simulink model "psm_sv_ekf_bemf_ctrl"  (R2026a)
settings: Solver=ode23tb  StopTime=simlength  FixedStep=tc  MaxStep=tc
values from neighbouring files (symbols this model uses):
  A1_tilde_ekf = [-Rs_norm/Lalpha_norm 0 0 0 0 0; 0 -Rs_norm/Lalpha_norm 0 0 0 0;      0 0 0 0 0 0; 0 0 0 0 0 0;      0 0 0 0 0 1; 0 0 0 0 0 0]    [kalman_psm.m]
  A2_tilde_ekf = [0 0 0 1/Lbeta_norm 0 0; 0 0 -1/Lbeta_norm 0 0 0;      0 0 0 -1 0 0; 0 0 1 0 0 0;     0 0 0 0 0 0; 0 0 0 0 0 0]    [kalman_psm.m]
  A3_tilde_ekf = [0 0 0 0 0 0; 0 0 0 0 0 -1/Lbeta_norm;      0 0 0 0 0 0; 0 0 0 0 0 1;     0 0 0 0 0 0; 0 0 0 0 0 0]    [kalman_psm.m]
  A4_tilde_ekf = [0 0 0 0 0 1/Lalpha_norm; 0 0 0 0 0 0;      0 0 0 0 0 -1; 0 0 0 0 0 0;     0 0 0 0 0 0; 0 0 0 0 0 0]    [kalman_psm.m]
  Bd_ekf = B_tilde_ekf*ts_inv    [kalman_psm.m]
  C_ekf = [1 0 0 0 0 0; 0 1 0 0 0 0]    [kalman_psm.m]
  CTRPIFF_CLIP_RELEASE = 0.001    [init_model.m]
  dead_time_INV = 3e-6    (= 3e-06)    [init_model.m]
  fPWM_INV = fPWM_AFE    (= 5000)    [init_model.m]
  g0_10Hz = fcut_10Hz_flt * ts_afe * 2*pi    (= 0.0125663706144)    [init_model.m]
  g0_1Hz = fcut_1Hz_flt * ts_afe * 2*pi    (= 0.00125663706144)    [init_model.m]
  g1_10Hz = 1 - g0_10Hz    (= 0.987433629386)    [init_model.m]
  g1_1Hz = 1 - g0_1Hz    (= 0.998743362939)    [init_model.m]
  id_lim = 0.35    [init_model.m]
  inv_m_scale = motorc_m_scale    [init_model.m]
  iq_lim = 1.4    [init_model.m]
  kg = Kobs(1)    [init_model.m]
  ki_align = 0.1    [init_model.m]
  ki_i = 18    [init_model.m]
  ki_w = 8    [init_model.m]
  kp_align = 0.6    [init_model.m]
  kp_i = 0.25    [init_model.m]
  kp_w = 2    [init_model.m]
  kw = Kobs(2)    [init_model.m]
  lim_down_align = -0.2    [init_model.m]
  lim_up_align = 0.2    [init_model.m]
  number_of_modules = 1    [init_model.m]
  omega_m_sim = omega_m_bez    [init_model.m]
  Qkalman = ts_inv * [Rs_norm/Lalpha_norm 0 0 0 0 0; 0 Rs_norm/Lbeta_norm 0 0 0 0;      0 0 1 0 0 0;     0 0 0 1 0 0;     0 0 0 0 1 0;     0 0 0 0 0 1]    [kalman_psm.m]
  Rkalman = [ts_inv 0; 0 ts_inv]    [kalman_psm.m]
  simlength = 2    [init_model.m]
  tc = ts_afe/100    (= 2e-06)    [init_model.m]
  time_gain_afe_module_1 = 1.0    (= 1)    [init_model.m]
  time_gain_inv_module_2 = 1.0    (= 1)    [init_model.m]
  time_start_motor_control = 0.025    [init_model.m]
  ts_inv = 1/fPWM_INV    (= 0.0002)    [init_model.m]
undefined symbols (not defined in the file or in its folder): ibez, La, Lb, Ld_norm, Lq_norm, magnitude, omega_bez, omega_m_bez, psi_bez, psi_m, rpm_base, rpm_bez, Rs, tau_bez, torque_base, ubez
libraries: fl_lib x24, nesl_utility x11, cstblocks_lti x2, single_phase_pwm_modulator x1, threephase_inductor_lib x1, simple_flexible_shaft x1, permanent_magnet_synchronous_machine x1
(part 2 of 2)

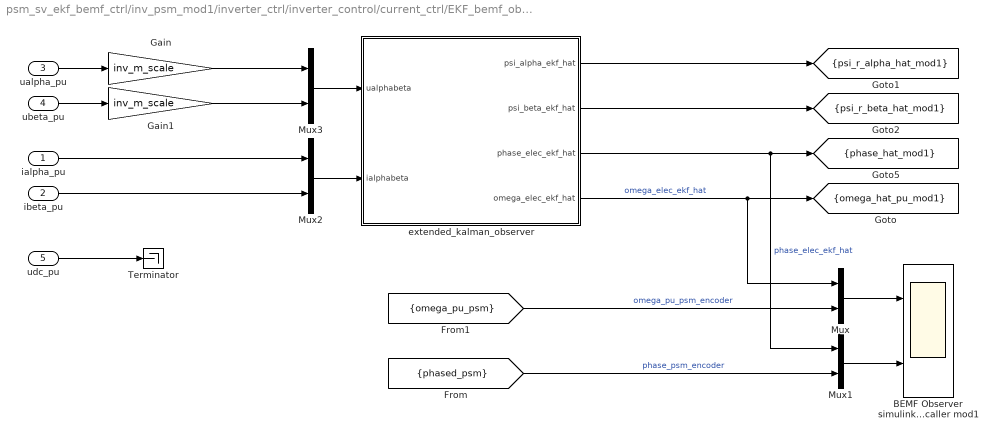
== system psm_sv_ekf_bemf_ctrl/inv_psm_mod1/inverter_ctrl/inverter_control/current_ctrl/EKF_bemf_observer ==
  ialpha_pu : Inport
  ibeta_pu : Inport  Port=2
  ualpha_pu : Inport  Port=3
  ubeta_pu : Inport  Port=4
  udc_pu : Inport  Port=5
  BEMF Observer simulink/Ccaller mod1 : Scope  NumInputPorts=2
      settings: ActiveDisplayYMinimum=-3.9268288357338932  ActiveDisplayYMaximum=3.9255329857071075
  Gain : Gain  Gain=inv_m_scale
  Gain1 : Gain  Gain=inv_m_scale
  Mux{,1..3} (4 alike) : Mux  Inputs=2
  Terminator : Terminator
  extended_kalman_observer : Subsystem
  tag scope: omega_hat_pu_mod1=scoped, phase_hat_mod1=scoped, psi_r_alpha_hat_mod1=scoped, psi_r_beta_hat_mod1=scoped
  wires:
  ialpha_pu/1 -> Mux2/1
  ibeta_pu/1 -> Mux2/2
  Mux/1 -> BEMF Observer simulink/Ccaller mod1/1
  Mux1/1 -> BEMF Observer simulink/Ccaller mod1/2
  ualpha_pu/1 -> Gain/1
  ubeta_pu/1 -> Gain1/1
  extended_kalman_observer/3(phase_elec_ekf_hat) -> [phase_hat_mod1], Mux1/1  "phase_elec_ekf_hat"
  extended_kalman_observer/4(omega_elec_ekf_hat) -> Mux/1, [omega_hat_pu_mod1]  "omega_elec_ekf_hat"
  [omega_pu_psm] -> Mux/2  "omega_pu_psm_encoder"
  [phased_psm] -> Mux1/2  "phase_psm_encoder"
  udc_pu/1 -> Terminator/1
  extended_kalman_observer/1(psi_alpha_ekf_hat) -> [psi_r_alpha_hat_mod1]
  extended_kalman_observer/2(psi_beta_ekf_hat) -> [psi_r_beta_hat_mod1]
  Mux2/1 -> extended_kalman_observer/2(ialphabeta)
  Mux3/1 -> extended_kalman_observer/1(ualphabeta)
  Gain/1 -> Mux3/1
  Gain1/1 -> Mux3/2

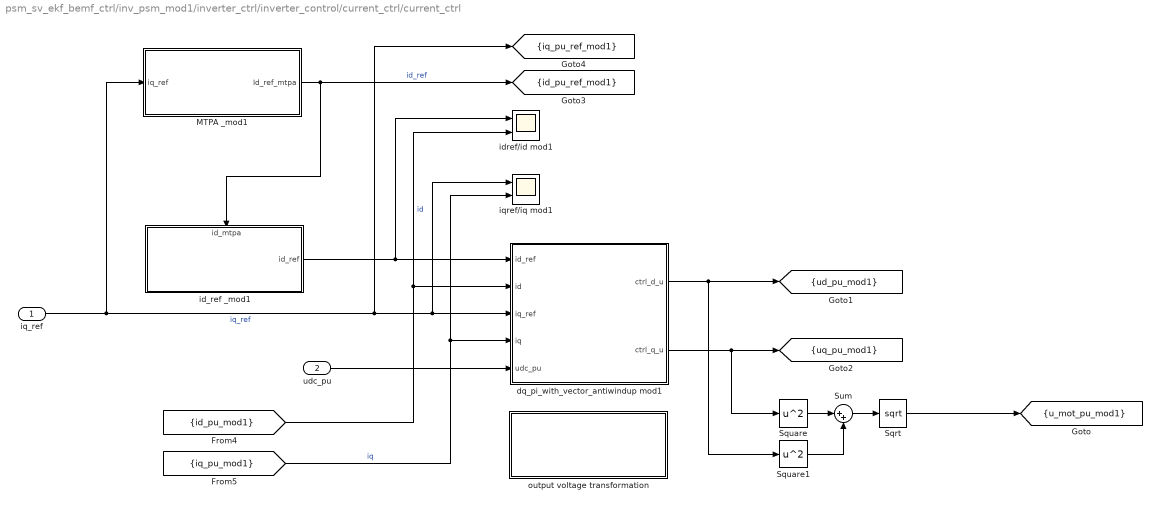
== system psm_sv_ekf_bemf_ctrl/inv_psm_mod1/inverter_ctrl/inverter_control/current_ctrl/current_ctrl ==
  iq_ref : Inport
  udc_pu : Inport  Port=2
  MTPA _mod1 : Subsystem
  Sqrt : Sqrt
  Square : Math  Operator=square
  Square1 : Math  Operator=square
  Sum : Sum  Inputs=|++
  dq_pi_with_vector_antiwindup mod1 : Subsystem
  id_ref _mod1 : Subsystem
      settings: PortSchema="{\"entries\":[{\"content\":{\"sides\":[{\"content\":{},\"type\":\"ConnectorPlacement.EquallySpacedRectSide\",\"uuid\":\"42af5d69-f0eb-42c6-9e03-28c1d0757323\"},{\"content\":{\"connectorIds\":[\"Out1\"],\"side\":\"RIGHT\"},\"type\":\"ConnectorPlacement.EquallySpacedRectSide\",\"uuid\":\"dd68a9f9-d15f-4e57-9d9e-130889a7b90c\"},{\"content\":{\"connectorIds\":[\"In1\"],\"side\":\"TOP\"},\"type\":\"ConnectorPlacement.EquallySpacedRectSide\",\"uuid\":\"68c797a2-8439-4b8d-8368-b7485adf0676\"}]},\"type\":\"ConnectorPlacement.EquallySpacedConnector\",\"uuid\":\"693c5f1c-0580-4626-8f13-b27865dfb3ac\"}],\"packageUris\":[\"http://schema.mathworks.com/mf0/Connector/R2020b\"],\"version\":\"1.0\"}"
  idref/id mod1 : Scope  NumInputPorts=2
      settings: ActiveDisplayYMinimum=-0.6792366431007606  ActiveDisplayYMaximum=0.075577635851628425
  iqref/iq mod1 : Scope  NumInputPorts=2
      settings: ActiveDisplayYMinimum=-2.4850184275737042  ActiveDisplayYMaximum=0.33436168402982208  DataLoggingVariableName=ScopeData2
  output voltage transformation : Subsystem
  tag scope: id_pu_ref_mod1=scoped, iq_pu_ref_mod1=scoped, u_mot_pu_mod1=scoped, ud_pu_mod1=scoped, uq_pu_mod1=scoped
  wires:
  [iq_pu_mod1] -> iqref/iq mod1/2, dq_pi_with_vector_antiwindup mod1/4(iq)  "iq"
  [id_pu_mod1] -> idref/id mod1/2, dq_pi_with_vector_antiwindup mod1/2(id)  "id"
  MTPA _mod1/1(Id_ref_mtpa) -> id_ref _mod1/1(id_mtpa), [id_pu_ref_mod1]  "id_ref"
  iq_ref/1 -> MTPA _mod1/1(iq_ref), iqref/iq mod1/1, dq_pi_with_vector_antiwindup mod1/3(iq_ref), [iq_pu_ref_mod1]  "iq_ref"
  dq_pi_with_vector_antiwindup mod1/1(ctrl_d_u) -> [ud_pu_mod1], Square1/1
  dq_pi_with_vector_antiwindup mod1/2(ctrl_q_u) -> [uq_pu_mod1], Square/1
  Square/1 -> Sum/1
  Sum/1 -> Sqrt/1
  Square1/1 -> Sum/2
  Sqrt/1 -> [u_mot_pu_mod1]
  id_ref _mod1/1(id_ref) -> idref/id mod1/1, dq_pi_with_vector_antiwindup mod1/1(id_ref)
  udc_pu/1 -> dq_pi_with_vector_antiwindup mod1/5(udc_pu)

== system psm_sv_ekf_bemf_ctrl/inv_psm_mod1/inverter_ctrl/inverter_control/current_ctrl/current_transformation ==
  Demux : Demux  Outputs=3
  alphabeta2dq : MATLAB Function  TreatAsAtomicUnit=on
  uvw2alphabeta : MATLAB Function  TreatAsAtomicUnit=on
  tag scope: ialpha_pu_mod1=scoped, ibeta_pu_mod1=scoped, id_pu_mod1=scoped, iq_pu_mod1=scoped
  wires:
  alphabeta2dq/2(q) -> [iq_pu_mod1]  "iq_pu"
  alphabeta2dq/1(d) -> [id_pu_mod1]  "id_pu"
  uvw2alphabeta/2(beta) -> alphabeta2dq/2(beta), [ibeta_pu_mod1]  "ibeta_pu"
  uvw2alphabeta/1(alpha) -> [ialpha_pu_mod1], alphabeta2dq/1(alpha)  "ialpha_pu"
  [motor_phase_ctrl_mod1] -> alphabeta2dq/3(gamma)
  Demux/3 -> uvw2alphabeta/3(w)  "iw"
  Demux/2 -> uvw2alphabeta/2(v)  "iv"
  Demux/1 -> uvw2alphabeta/1(u)  "iu"
  [isd_uvw_inv_mod1] -> Demux/1

== system psm_sv_ekf_bemf_ctrl/inv_psm_mod1/inverter_ctrl/inverter_control/encoder-sensorless-switch/double_integrator_observer ==
  phase_psm : Inport
  Dead Zone : DeadZone  LowerValue=-0.01  UpperValue=0.01
  Gain : Gain  Gain=kw
  Gain1 : Gain  Gain=kg
  Gain2 : Gain  Gain=omega_bez
  Gain3 : Gain  Gain=1/omega_bez
  Gain5 : Gain  Gain=ts_inv
  Sum : Sum  Inputs=-+|
  Sum1 : Sum  Inputs=|++
  Sum2 : Sum  Inputs=|++
  Sum8 : Sum  Inputs=++|
  Unit Delay1 : UnitDelay  InitialCondition=pi  SampleTime=-1
  Unit Delay2 : UnitDelay  SampleTime=-1
  bounder1 : MATLAB Function  TreatAsAtomicUnit=on
  bounder2 : MATLAB Function  TreatAsAtomicUnit=on
  phase_psm_hat : Outport  VectorParamsAs1DForOutWhenUnconnected=off
  omega_pu_psm_hat : Outport  Port=2  VectorParamsAs1DForOutWhenUnconnected=off
  wires:
  Gain1/1 -> Sum2/1
  phase_psm/1 -> Sum/2
  Sum8/1 -> Unit Delay1/1
  Unit Delay1/1 -> bounder2/1(u)
  Sum1/1 -> Unit Delay2/1
  Gain/1 -> Gain3/1
  Unit Delay2/1 -> omega_pu_psm_hat/1, Sum1/2, Gain5/1
  Sum2/1 -> Sum8/2
  bounder2/1(y) -> Sum2/2, phase_psm_hat/1, Sum/1  "phase_hat"
  bounder1/1(y) -> Gain1/1, Gain/1
  Gain2/1 -> Sum8/1
  Gain3/1 -> Sum1/1
  Gain5/1 -> Gain2/1
  Sum/1 -> bounder1/1(u)

== system psm_sv_ekf_bemf_ctrl/inv_psm_mod1/inverter_ctrl/inverter_control/is inv quantizzation and one step delay/is inv quantizzation and one step delay ==
  is_u_pu : Inport
  is_v_pu : Inport  Port=2
  is_w_pu : Inport  Port=3
  Gain3 : Gain  Gain=-1
  Gain4 : Gain  Gain=-1
  Gain5 : Gain  Gain=-1
  Quantizer : Quantizer  QuantizationInterval=adc_quantization
  Quantizer1 : Quantizer  QuantizationInterval=adc_quantization
  Quantizer2 : Quantizer  QuantizationInterval=adc_quantization
  Unit Delay : UnitDelay  SampleTime=-1
  Unit Delay1 : UnitDelay  SampleTime=-1
  Unit Delay2 : UnitDelay  SampleTime=-1
  Zero-Order Hold : ZeroOrderHold  SampleTime=-1
  Zero-Order Hold1 : ZeroOrderHold  SampleTime=-1
  Zero-Order Hold2 : ZeroOrderHold  SampleTime=-1
  isd_u_pu : Outport
  isd_v_pu : Outport  Port=2
  isd_w_pu : Outport  Port=3
  wires:
  Unit Delay/1 -> Gain3/1
  Unit Delay1/1 -> Gain4/1
  Unit Delay2/1 -> Gain5/1
  Quantizer/1 -> Unit Delay/1
  Quantizer1/1 -> Unit Delay1/1
  Quantizer2/1 -> Unit Delay2/1
  is_u_pu/1 -> Zero-Order Hold/1
  is_v_pu/1 -> Zero-Order Hold1/1
  is_w_pu/1 -> Zero-Order Hold2/1
  Gain3/1 -> isd_u_pu/1
  Gain4/1 -> isd_v_pu/1
  Gain5/1 -> isd_w_pu/1
  Zero-Order Hold/1 -> Quantizer/1
  Zero-Order Hold1/1 -> Quantizer1/1
  Zero-Order Hold2/1 -> Quantizer2/1

== system psm_sv_ekf_bemf_ctrl/inv_psm_mod1/inverter_ctrl/inverter_control/omega_pu/flt ==
  input : Inport
  Gain3 : Gain  Gain=g1_10Hz
  Gain6 : Gain  Gain=g0_10Hz
  Sum : Sum  Inputs=|++
  Unit Delay1 : UnitDelay  SampleTime=-1
  output : Outport  VectorParamsAs1DForOutWhenUnconnected=off
  wires:
  Gain6/1 -> Sum/1
  input/1 -> Gain6/1
  Unit Delay1/1 -> Gain3/1
  Gain3/1 -> Sum/2
  Sum/1 -> Unit Delay1/1, output/1

== system psm_sv_ekf_bemf_ctrl/inv_psm_mod1/inverter_ctrl/inverter_control/phase_compensation_1/alignment_ctrl ==
  local_time : Inport
  master_time : Inport  Port=2
  Constant : Constant  Value=0
  Gain : Gain  Gain=-1
  Sum : Sum  Inputs=|+-
  pi : Subsystem  mask{kp=kp_align, ki=ki_align, lim_up=lim_up_align, lim_down=lim_down_align}
      mask prompts: ki "ki*ts"
      mask Display:
      | disp('pi()');
      | port_label('input', 1, 'u_ref');
      | port_label('input', 2, 'u');
      | port_label('output', 1, 'y');
  dp : Outport
  wires:
  master_time/1 -> Sum/1
  Sum/1 -> Gain/1
  Constant/1 -> pi/1(u_ref)
  local_time/1 -> Sum/2
  Gain/1 -> pi/2(u)
  pi/1(y) -> dp/1

== system psm_sv_ekf_bemf_ctrl/inv_psm_mod1/inverter_ctrl/inverter_control/speed_reference_generator/flt ==
  input : Inport
  Gain3 : Gain  Gain=g1_1Hz
  Gain6 : Gain  Gain=g0_1Hz
  Sum : Sum  Inputs=|++
  Unit Delay1 : UnitDelay  SampleTime=-1
  output : Outport  VectorParamsAs1DForOutWhenUnconnected=off
  wires:
  Gain6/1 -> Sum/1
  input/1 -> Gain6/1
  Unit Delay1/1 -> Gain3/1
  Gain3/1 -> Sum/2
  Sum/1 -> Unit Delay1/1, output/1

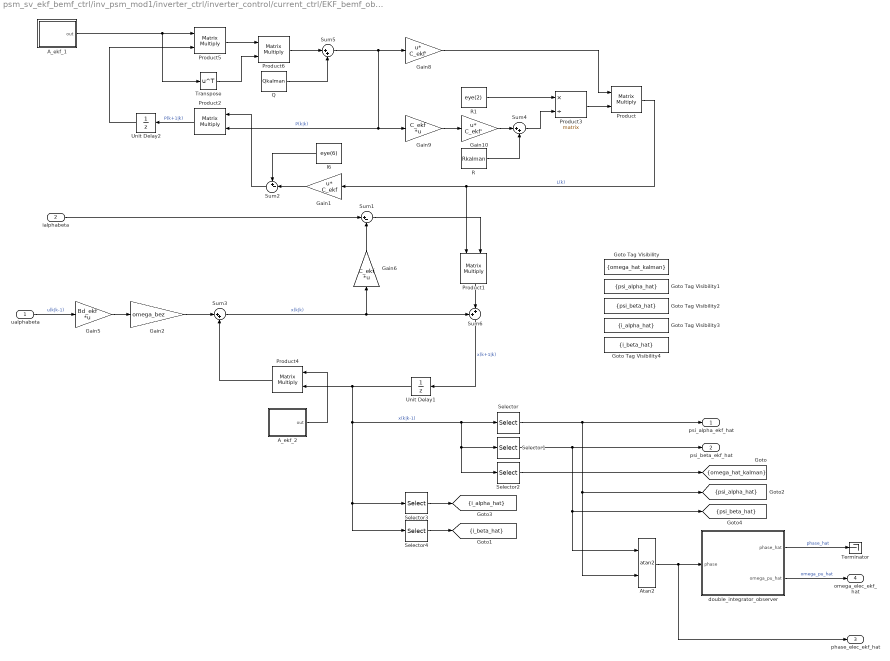
== system psm_sv_ekf_bemf_ctrl/inv_psm_mod1/inverter_ctrl/inverter_control/current_ctrl/EKF_bemf_observer/extended_kalman_observer ==
  ualphabeta : Inport
  ialphabeta : Inport  Port=2
  A_ekf_1 : Subsystem
  A_ekf_2 : Subsystem
  Atan2 : Trigonometry  Operator=atan2
  Gain1 : Gain  Gain=C_ekf  Multiplication=Matrix(u*K)
  Gain10 : Gain  Gain=C_ekf'  Multiplication=Matrix(u*K)
  Gain2 : Gain  Gain=omega_bez
  Gain5 : Gain  Gain=Bd_ekf  Multiplication=Matrix(K*u)
  Gain6 : Gain  Gain=C_ekf  Multiplication=Matrix(K*u)
  Gain8 : Gain  Gain=C_ekf'  Multiplication=Matrix(u*K)
  Gain9 : Gain  Gain=C_ekf  Multiplication=Matrix(K*u)
  Goto Tag Visibility : GotoTagVisibility  GotoTag=omega_hat_kalman
  Goto Tag Visibility1 : GotoTagVisibility  GotoTag=psi_alpha_hat
  Goto Tag Visibility2 : GotoTagVisibility  GotoTag=psi_beta_hat
  Goto Tag Visibility3 : GotoTagVisibility  GotoTag=i_alpha_hat
  Goto Tag Visibility4 : GotoTagVisibility  GotoTag=i_beta_hat
  I6 : Constant  Value=eye(6)
  Product{,1..2,4..6} (6 alike) : Product  Multiplication=Matrix(*)
  Product3 : Product  Inputs=*/  Multiplication=Matrix(*)
  Q : Constant  Value=Qkalman
  R : Constant  Value=Rkalman
  R1 : Constant  Value=eye(2)
  Selector : Selector  InputPortWidth=6  IndexOptions=Index vector (dialog)  Indices=3  OutputSizes=1
  Selector1 : Selector  InputPortWidth=6  IndexOptions=Index vector (dialog)  Indices=4  OutputSizes=1
  Selector2 : Selector  InputPortWidth=6  IndexOptions=Index vector (dialog)  Indices=6  OutputSizes=1
  Selector3 : Selector  InputPortWidth=6  IndexOptions=Index vector (dialog)  Indices=1  OutputSizes=1
  Selector4 : Selector  InputPortWidth=6  IndexOptions=Index vector (dialog)  Indices=2  OutputSizes=1
  Sum1 : Sum  Inputs=|+-
  Sum2 : Sum  Inputs=+-|
  Sum3 : Sum  Inputs=|++
  Sum4 : Sum  Inputs=|++
  Sum5 : Sum  Inputs=|++
  Sum6 : Sum  Inputs=++|
  Terminator : Terminator
  Transpose : Math  Operator=transpose
  Unit Delay1 : UnitDelay  InitialCondition=[0 0 1 1 0 0]*ts_inv  SampleTime=-1
  Unit Delay2 : UnitDelay  SampleTime=-1
  double_integrator_observer : Subsystem
  psi_alpha_ekf_hat : Outport
  psi_beta_ekf_hat : Outport  Port=2
  phase_elec_ekf_hat : Outport  Port=3
  omega_elec_ekf_hat : Outport  Port=4
  tag scope: i_alpha_hat=scoped, i_beta_hat=scoped, omega_hat_kalman=scoped, psi_alpha_hat=scoped, psi_beta_hat=scoped
  wires:
  Gain5/1 -> Gain2/1
  Gain6/1 -> Sum1/2
  Sum5/1 -> Gain8/1, Gain9/1, Product2/2  "P(k|k)"
  Product5/1 -> Product6/1
  Product6/1 -> Sum5/1
  Q/1 -> Sum5/2
  Gain9/1 -> Gain10/1
  R/1 -> Sum4/2
  Gain10/1 -> Sum4/1
  Gain8/1 -> Product/1
  Product/1 -> Product1/1, Gain1/1  "L(k)"
  Product2/1 -> Unit Delay2/1  "P(k+1|k)"
  Sum2/1 -> Product2/1
  Unit Delay2/1 -> Product5/2
  Sum6/1 -> Unit Delay1/1  "x(k+1|k)"
  I6/1 -> Sum2/1
  Gain1/1 -> Sum2/2
  Sum1/1 -> Product1/2
  ialphabeta/1 -> Sum1/1
  Sum4/1 -> Product3/2
  Product3/1 -> Product/2
  R1/1 -> Product3/1
  ualphabeta/1 -> Gain5/1  "u(k|k-1)"
  Sum3/1 -> Gain6/1, Sum6/1  "x(k|k)"
  Unit Delay1/1 -> Selector2/1, Selector1/1, Selector/1, Selector3/1, Selector4/1, Product4/2  "x(k|k-1)"
  A_ekf_2/1(out) -> Product4/1
  A_ekf_1/1(out) -> Transpose/1, Product5/1
  Product1/1 -> Sum6/2
  Selector1/1 -> Atan2/1, [psi_beta_hat], psi_beta_ekf_hat/1
  Selector/1 -> Atan2/2, [psi_alpha_hat], psi_alpha_ekf_hat/1
  Transpose/1 -> Product6/2
  Selector2/1 -> [omega_hat_kalman]
  Selector3/1 -> [i_alpha_hat]
  Selector4/1 -> [i_beta_hat]
  Product4/1 -> Sum3/2
  double_integrator_observer/2(omega_pu_hat) -> omega_elec_ekf_hat/1  "omega_pu_hat"
  Atan2/1 -> double_integrator_observer/1(phase), phase_elec_ekf_hat/1
  double_integrator_observer/1(phase_hat) -> Terminator/1  "phase_hat"
  Gain2/1 -> Sum3/1

== system psm_sv_ekf_bemf_ctrl/inv_psm_mod1/inverter_ctrl/inverter_control/current_ctrl/current_ctrl/MTPA _mod1 ==
  iq_ref : Inport
  Gain1 : Gain  Gain=1/(Ld_norm - Lq_norm)/2
  Gain2 : Gain  Gain=1/(Ld_norm - Lq_norm)/2
  Gain3 : Gain  Gain=-1
  Math Function1 : Math  Operator=magnitude^2  SignedPower=on
  Math Function4 : Math  Operator=magnitude^2  SignedPower=on
  Sqrt : Sqrt
  Sum : Sum  Inputs=|++
  Sum1 : Sum  Inputs=|-+
  id_ref_pu < x < 0 : Saturate  UpperLimit=0  LowerLimit=-id_lim
  Id_ref_mtpa : Outport  VectorParamsAs1DForOutWhenUnconnected=off
  wires:
  Sum1/1 -> Gain3/1
  id_ref_pu < x < 0/1 -> Id_ref_mtpa/1
  Math Function4/1 -> Sum/1
  Math Function1/1 -> Sum/2
  Gain1/1 -> Math Function4/1
  Sum/1 -> Sqrt/1
  Sqrt/1 -> Sum1/2
  iq_ref/1 -> Math Function1/1
  Gain2/1 -> Sum1/1
  [motor_speed_pu_ctrl_mod1] -> Gain1/1, Gain2/1
  Gain3/1 -> id_ref_pu < x < 0/1

== system psm_sv_ekf_bemf_ctrl/inv_psm_mod1/inverter_ctrl/inverter_control/current_ctrl/current_ctrl/dq_pi_with_vector_antiwindup mod1 ==
  id_ref : Inport
  id : Inport  Port=2
  iq_ref : Inport  Port=3
  iq : Inport  Port=4
  udc_pu : Inport  Port=5
  Variant Source : VariantSource  VariantControls={use_current_controller_from_simulink_module_1 == 1, use_current_controller_from_ccaller_module_1 == 1}
  Variant Source1 : VariantSource  VariantControls={use_current_controller_from_simulink_module_1 == 1, use_current_controller_from_ccaller_module_1 == 1}
  dq_vector_pi : Subsystem
  dq_vector_pi_ccaller : Subsystem
  simulink/Ccaller VectorPI : Scope  NumInputPorts=2
      settings: ActiveDisplayYMinimum=-1.0778845462482423  ActiveDisplayYMaximum=0.14052729005925355
  ctrl_d_u : Outport
  ctrl_q_u : Outport  Port=2
  wires:
  id/1 -> dq_vector_pi_ccaller/1(id), dq_vector_pi/1(id)  "id"
  id_ref/1 -> dq_vector_pi_ccaller/2(id_ref), dq_vector_pi/2(id_ref)  "id_ref"
  iq/1 -> dq_vector_pi_ccaller/3(iq), dq_vector_pi/3(iq)  "iq"
  iq_ref/1 -> dq_vector_pi_ccaller/4(iq_ref), dq_vector_pi/4(iq_ref)  "iq_ref"
  dq_vector_pi/1(md_sat) -> Variant Source/1
  dq_vector_pi_ccaller/2(uq_ctrl_out) -> Variant Source1/2
  dq_vector_pi/2(mq_sat) -> Variant Source1/1
  dq_vector_pi_ccaller/1(ud_ctrl_out) -> Variant Source/2
  Variant Source/1 -> ctrl_d_u/1, simulink/Ccaller VectorPI/1  "ctrl_d_u"
  Variant Source1/1 -> simulink/Ccaller VectorPI/2, ctrl_q_u/1  "ctrl_q_u"
  udc_pu/1 -> dq_vector_pi_ccaller/5(udc_pu)

== system psm_sv_ekf_bemf_ctrl/inv_psm_mod1/inverter_ctrl/inverter_control/current_ctrl/current_ctrl/id_ref _mod1 ==
  id_mtpa : Inport
  Constant : Constant  Value=0
  Variant Source : VariantSource  VariantControls={use_mtpa == 1, use_mtpa == 0}
  id_ref : Outport
  wires:
  Variant Source/1 -> id_ref/1
  id_mtpa/1 -> Variant Source/1
  Constant/1 -> Variant Source/2

== system psm_sv_ekf_bemf_ctrl/inv_psm_mod1/inverter_ctrl/inverter_control/current_ctrl/current_ctrl/output voltage transformation ==
  Unit Delay2 : UnitDelay  SampleTime=-1
  Unit Delay3 : UnitDelay  SampleTime=-1
  dq2alphabeta : MATLAB Function  TreatAsAtomicUnit=on
  tag scope: ualpha_pu_mod1=scoped, ubeta_pu_mod1=scoped
  wires:
  [ud_pu_mod1] -> dq2alphabeta/1(d)
  [uq_pu_mod1] -> dq2alphabeta/2(q)
  Unit Delay2/1 -> [ualpha_pu_mod1]
  dq2alphabeta/2(beta) -> Unit Delay3/1
  Unit Delay3/1 -> [ubeta_pu_mod1]
  dq2alphabeta/1(alpha) -> Unit Delay2/1
  [motor_phase_ctrl_mod1] -> dq2alphabeta/3(gamma)

== system psm_sv_ekf_bemf_ctrl/inv_psm_mod1/inverter_ctrl/inverter_control/phase_compensation_1/alignment_ctrl/pi ==
  u_ref : Inport
  u : Inport  Port=2
  1/Ti : Gain  Gain=kp  SaturateOnIntegerOverflow=on  OutDataTypeStr=Inherit: Same as input  ParamDataTypeStr=Inherit: Same as input
  Saturation : Saturate  UpperLimit=lim_up  LowerLimit=lim_down
  Sum1 : Sum  Inputs=+++  SaturateOnIntegerOverflow=on
  Sum2 : Sum  Inputs=-+  SaturateOnIntegerOverflow=on
  Sum3 : Sum  Inputs=-+  SaturateOnIntegerOverflow=on
  Unit Delay4 : UnitDelay  SampleTime=-1
  kp : Gain  Gain=ki  SaturateOnIntegerOverflow=on  OutDataTypeStr=Inherit: Same as input  ParamDataTypeStr=Inherit: Same as input
  y : Outport
  wires:
  1/Ti/1 -> Sum1/1, Sum3/1
  kp/1 -> Sum1/2
  Sum3/1 -> Unit Delay4/1
  Unit Delay4/1 -> Sum1/3
  u_ref/1 -> Sum2/2
  u/1 -> Sum2/1
  Sum2/1 -> kp/1, 1/Ti/1
  Sum1/1 -> Saturation/1
  Saturation/1 -> Sum3/2, y/1

== system psm_sv_ekf_bemf_ctrl/inv_psm_mod1/inverter_ctrl/inverter_control/current_ctrl/EKF_bemf_observer/extended_kalman_observer/A_ekf_1 ==
  Gain1 : Gain  Gain=A2_tilde_ekf
  Gain{7..10} (4 alike) : Gain  Gain=omega_bez
  Gain{2,4,6,11} (4 alike) : Gain  Gain=ts_inv
  Gain3 : Gain  Gain=A3_tilde_ekf
  Gain5 : Gain  Gain=A4_tilde_ekf
  I1 : Constant  Value=eye(6)
  I2 : Constant  Value=A1_tilde_ekf
  Sum7 : Sum  Inputs=+++++
  out : Outport
  wires:
  [psi_beta_hat] -> Gain5/1
  [psi_alpha_hat] -> Gain3/1
  [omega_hat_kalman] -> Gain1/1
  Gain5/1 -> Gain6/1
  Gain3/1 -> Gain4/1
  Gain1/1 -> Gain2/1
  I1/1 -> Sum7/1
  I2/1 -> Gain11/1
  Sum7/1 -> out/1
  Gain11/1 -> Gain7/1
  Gain2/1 -> Gain8/1
  Gain4/1 -> Gain9/1
  Gain6/1 -> Gain10/1
  Gain7/1 -> Sum7/2
  Gain8/1 -> Sum7/3
  Gain9/1 -> Sum7/4
  Gain10/1 -> Sum7/5

== system psm_sv_ekf_bemf_ctrl/inv_psm_mod1/inverter_ctrl/inverter_control/current_ctrl/EKF_bemf_observer/extended_kalman_observer/A_ekf_2 ==
  Gain1 : Gain  Gain=A2_tilde_ekf
  Gain{7..10} (4 alike) : Gain  Gain=omega_bez
  Gain{2,4,6,11} (4 alike) : Gain  Gain=ts_inv
  Gain3 : Gain  Gain=A3_tilde_ekf
  Gain5 : Gain  Gain=A4_tilde_ekf
  I1 : Constant  Value=eye(6)
  I2 : Constant  Value=A1_tilde_ekf
  Sum7 : Sum  Inputs=+++++
  out : Outport
  wires:
  Sum7/1 -> out/1
  I2/1 -> Gain11/1
  I1/1 -> Sum7/1
  Gain1/1 -> Gain2/1
  Gain3/1 -> Gain4/1
  Gain5/1 -> Gain6/1
  [omega_hat_kalman] -> Gain1/1
  [psi_alpha_hat] -> Gain3/1
  [psi_beta_hat] -> Gain5/1
  Gain11/1 -> Gain7/1
  Gain2/1 -> Gain8/1
  Gain4/1 -> Gain9/1
  Gain6/1 -> Gain10/1
  Gain7/1 -> Sum7/2
  Gain8/1 -> Sum7/3
  Gain9/1 -> Sum7/4
  Gain10/1 -> Sum7/5

== system psm_sv_ekf_bemf_ctrl/inv_psm_mod1/inverter_ctrl/inverter_control/current_ctrl/EKF_bemf_observer/extended_kalman_observer/double_integrator_observer ==
  phase : Inport
  Dead Zone : DeadZone  LowerValue=-0.01  UpperValue=0.01
  Gain : Gain  Gain=kw
  Gain1 : Gain  Gain=kg
  Gain2 : Gain  Gain=omega_bez
  Gain3 : Gain  Gain=1/omega_bez
  Gain5 : Gain  Gain=ts_inv
  Sum : Sum  Inputs=-+|
  Sum1 : Sum  Inputs=|++
  Sum2 : Sum  Inputs=|++
  Sum8 : Sum  Inputs=++|
  Unit Delay1 : UnitDelay  InitialCondition=pi  SampleTime=-1
  Unit Delay2 : UnitDelay  SampleTime=-1
  bounder1 : MATLAB Function  TreatAsAtomicUnit=on
  bounder2 : MATLAB Function  TreatAsAtomicUnit=on
  phase_hat : Outport  VectorParamsAs1DForOutWhenUnconnected=off
  omega_pu_hat : Outport  Port=2  VectorParamsAs1DForOutWhenUnconnected=off
  wires:
  Gain1/1 -> Sum2/1
  phase/1 -> Sum/2
  Sum8/1 -> Unit Delay1/1
  Unit Delay1/1 -> bounder2/1(u)
  Sum1/1 -> Unit Delay2/1
  Gain/1 -> Gain3/1
  Unit Delay2/1 -> omega_pu_hat/1, Sum1/2, Gain5/1
  Sum2/1 -> Sum8/2
  bounder2/1(y) -> Sum2/2, phase_hat/1, Sum/1  "phase_hat"
  bounder1/1(y) -> Gain1/1, Gain/1
  Gain2/1 -> Sum8/1
  Gain3/1 -> Sum1/1
  Gain5/1 -> Gain2/1
  Sum/1 -> bounder1/1(u)

== system psm_sv_ekf_bemf_ctrl/inv_psm_mod1/inverter_ctrl/inverter_control/current_ctrl/current_ctrl/dq_pi_with_vector_antiwindup mod1/dq_vector_pi ==
  id : Inport
  id_ref : Inport  Port=2
  iq : Inport  Port=3
  iq_ref : Inport  Port=4
  Sum1 : Sum  Inputs=|-+
  Sum2 : Sum  Inputs=|-+
  bounder1 : Subsystem
  bounder2 : Subsystem
  pi_d : Subsystem
  pi_q : Subsystem
  switch : Subsystem
  vector lenght : Subsystem
  md_sat : Outport
  mq_sat : Outport  Port=2
  wires:
  bounder2/2(clip) -> switch/2(clip 2)
  vector lenght/2(m) -> bounder1/3(m), bounder2/1(m)
  Sum2/1 -> pi_q/1(iq_tilde)
  pi_d/1(ud_out) -> vector lenght/1(md), bounder1/1(md)
  pi_q/1(Vqs_out) -> bounder2/3(mq), vector lenght/2(mq)
  vector lenght/1(m_1) -> bounder1/2(m_1), bounder2/2(m_1)
  switch/1(clip) -> pi_q/2(clip), pi_d/2(clip)
  iq/1 -> Sum2/1
  Sum1/1 -> pi_d/1(id_tilde)
  bounder1/2(clip) -> switch/1(clip 1)
  id/1 -> Sum1/1
  bounder1/1(md_sat) -> md_sat/1
  bounder2/1(mq_sat) -> mq_sat/1
  id_ref/1 -> Sum1/2
  iq_ref/1 -> Sum2/2

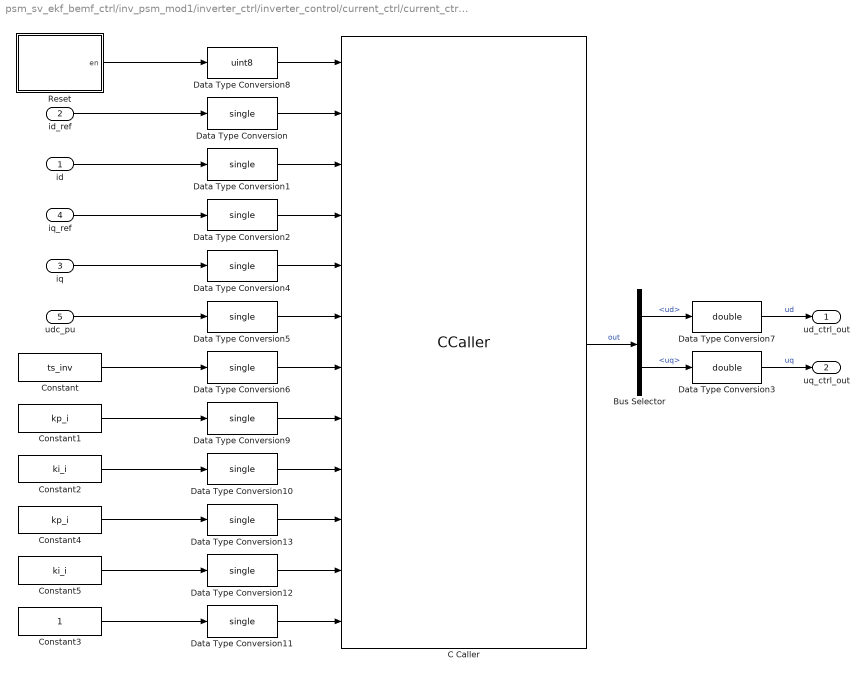
== system psm_sv_ekf_bemf_ctrl/inv_psm_mod1/inverter_ctrl/inverter_control/current_ctrl/current_ctrl/dq_pi_with_vector_antiwindup mod1/dq_vector_pi_ccaller ==
  id : Inport
  id_ref : Inport  Port=2
  iq : Inport  Port=3
  iq_ref : Inport  Port=4
  udc_pu : Inport  Port=5
  Bus Selector : BusSelector  OutputSignals=ud,uq
  C Caller : CCaller  FunctionName=dqvector_pi_process_simulink  PortSpecificationStruct="%)30     .    ,!8   8    (     @         %    \"     T    !     0         %  0 \"0    $    _    07)G3F%M90  4&]R=$YA;64 4V-O<&4     26YD97@     5'EP90      4VEZ90      27-';&]B86P   X    P    !@    @    $          4    (     0    ,    !         !   P!O=70 #@   #     &    \"     0         !0    @    !     P    $         $  # &]U=  .    .     8    (    !          %    \"     $    &     0         0   ...(+7280 chars)"
  Constant : Constant  Value=ts_inv
  Constant1 : Constant  Value=kp_i
  Constant2 : Constant  Value=ki_i
  Constant3 : Constant
  Constant4 : Constant  Value=kp_i
  Constant5 : Constant  Value=ki_i
  Data Type Conversion{,1..2,4..6,9..13} (11 alike) : DataTypeConversion  OutDataTypeStr=single  SaturateOnIntegerOverflow=off  RndMeth=Floor
  Data Type Conversion3 : DataTypeConversion  OutDataTypeStr=double  SaturateOnIntegerOverflow=off  RndMeth=Floor
  Data Type Conversion7 : DataTypeConversion  OutDataTypeStr=double  SaturateOnIntegerOverflow=off  RndMeth=Floor
  Data Type Conversion8 : DataTypeConversion  OutDataTypeStr=uint8  SaturateOnIntegerOverflow=off  RndMeth=Floor
  Reset : Subsystem
  ud_ctrl_out : Outport
  uq_ctrl_out : Outport  Port=2
  wires:
  Data Type Conversion5/1 -> C Caller/6
  Data Type Conversion/1 -> C Caller/2
  C Caller/1 -> Bus Selector/1  "out"
  Data Type Conversion1/1 -> C Caller/3
  Data Type Conversion4/1 -> C Caller/5
  Data Type Conversion2/1 -> C Caller/4
  Data Type Conversion6/1 -> C Caller/7
  Bus Selector/2 -> Data Type Conversion3/1  "<uq>"
  Bus Selector/1 -> Data Type Conversion7/1  "<ud>"
  Data Type Conversion7/1 -> ud_ctrl_out/1  "ud"
  Data Type Conversion3/1 -> uq_ctrl_out/1  "uq"
  Data Type Conversion8/1 -> C Caller/1
  Data Type Conversion9/1 -> C Caller/8
  Data Type Conversion10/1 -> C Caller/9
  Data Type Conversion11/1 -> C Caller/12
  Data Type Conversion13/1 -> C Caller/10
  Data Type Conversion12/1 -> C Caller/11
  Constant3/1 -> Data Type Conversion11/1
  Constant5/1 -> Data Type Conversion12/1
  Constant4/1 -> Data Type Conversion13/1
  Constant2/1 -> Data Type Conversion10/1
  Constant1/1 -> Data Type Conversion9/1
  Constant/1 -> Data Type Conversion6/1
  udc_pu/1 -> Data Type Conversion5/1
  iq/1 -> Data Type Conversion4/1
  iq_ref/1 -> Data Type Conversion2/1
  Reset/1(en) -> Data Type Conversion8/1
  id_ref/1 -> Data Type Conversion/1
  id/1 -> Data Type Conversion1/1

== system psm_sv_ekf_bemf_ctrl/inv_psm_mod1/inverter_ctrl/inverter_control/current_ctrl/current_ctrl/dq_pi_with_vector_antiwindup mod1/dq_vector_pi/bounder1 ==
  md : Inport
  m_1 : Inport  Port=2
  m : Inport  Port=3
  Constant : Constant
  Constant1 : Constant  Value=0
  Divide : Product
  Switch : Switch  Threshold=1  SaturateOnIntegerOverflow=off  InputSameDT=off
  Switch1 : Switch  Threshold=1  SaturateOnIntegerOverflow=off  InputSameDT=off
  md_sat : Outport  VectorParamsAs1DForOutWhenUnconnected=off
  clip : Outport  Port=2  VectorParamsAs1DForOutWhenUnconnected=off
  wires:
  md/1 -> Switch1/3, Divide/2
  m_1/1 -> Divide/1
  Divide/1 -> Switch1/1
  Switch1/1 -> md_sat/1
  Switch/1 -> clip/1
  m/1 -> Switch/2, Switch1/2
  Constant/1 -> Switch/1
  Constant1/1 -> Switch/3

== system psm_sv_ekf_bemf_ctrl/inv_psm_mod1/inverter_ctrl/inverter_control/current_ctrl/current_ctrl/dq_pi_with_vector_antiwindup mod1/dq_vector_pi/bounder2 ==
  m : Inport
  m_1 : Inport  Port=2
  mq : Inport  Port=3
  Constant : Constant
  Constant1 : Constant  Value=0
  Divide : Product
  Switch : Switch  Threshold=1  SaturateOnIntegerOverflow=off  InputSameDT=off
  Switch1 : Switch  Threshold=1  SaturateOnIntegerOverflow=off  InputSameDT=off
  mq_sat : Outport  VectorParamsAs1DForOutWhenUnconnected=off
  clip : Outport  Port=2  VectorParamsAs1DForOutWhenUnconnected=off
  wires:
  Constant1/1 -> Switch/3
  Constant/1 -> Switch/1
  m/1 -> Switch1/2, Switch/2
  Switch/1 -> clip/1
  Switch1/1 -> mq_sat/1
  Divide/1 -> Switch1/1
  m_1/1 -> Divide/1
  mq/1 -> Divide/2, Switch1/3

== system psm_sv_ekf_bemf_ctrl/inv_psm_mod1/inverter_ctrl/inverter_control/current_ctrl/current_ctrl/dq_pi_with_vector_antiwindup mod1/dq_vector_pi/pi_d ==
  id_tilde : Inport
  clip : Inport  Port=2
  1/Ti : Gain  Gain=kp_i  SaturateOnIntegerOverflow=on  OutDataTypeStr=Inherit: Same as input  ParamDataTypeStr=Inherit: Same as input
  Constant : Constant  Value=0
  Sum2 : Sum  Inputs=+-  SaturateOnIntegerOverflow=on
  Sum4 : Sum  SaturateOnIntegerOverflow=on
  Sum5 : Sum  SaturateOnIntegerOverflow=on
  Switch1 : Switch  Threshold=0.5  SaturateOnIntegerOverflow=off  InputSameDT=off
  Switch2 : Switch  Threshold=0.5  SaturateOnIntegerOverflow=off  InputSameDT=off
  Unit Delay1 : UnitDelay  SampleTime=-1
  Unit Delay2 : UnitDelay  SampleTime=-1
  kp1 : Gain  Gain=CTRPIFF_CLIP_RELEASE*ts_inv  SaturateOnIntegerOverflow=on  OutDataTypeStr=Inherit: Same as input  ParamDataTypeStr=Inherit: Same as input
  kp2 : Gain  Gain=ki_i*ts_inv  SaturateOnIntegerOverflow=on  OutDataTypeStr=Inherit: Same as input  ParamDataTypeStr=Inherit: Same as input
  ud_out : Outport  VectorParamsAs1DForOutWhenUnconnected=off
  wires:
  id_tilde/1 -> kp2/1, 1/Ti/1
  Sum5/1 -> ud_out/1
  Switch1/1 -> Unit Delay2/1
  Sum4/1 -> Sum5/2, Switch1/3
  kp1/1 -> Sum2/2
  Sum2/1 -> Switch1/1
  Unit Delay2/1 -> Sum4/2, kp1/1, Sum2/1
  1/Ti/1 -> Sum5/1
  Switch2/1 -> Sum4/1
  kp2/1 -> Switch2/3
  clip/1 -> Unit Delay1/1
  [clip] -> Switch2/2
  [clip] -> Switch1/2
  Constant/1 -> Switch2/1
  Unit Delay1/1 -> [clip]

== system psm_sv_ekf_bemf_ctrl/inv_psm_mod1/inverter_ctrl/inverter_control/current_ctrl/current_ctrl/dq_pi_with_vector_antiwindup mod1/dq_vector_pi/pi_q ==
  iq_tilde : Inport
  clip : Inport  Port=2
  1/Ti : Gain  Gain=kp_i  SaturateOnIntegerOverflow=on  OutDataTypeStr=Inherit: Same as input  ParamDataTypeStr=Inherit: Same as input
  Constant : Constant  Value=0
  Sum2 : Sum  Inputs=+-  SaturateOnIntegerOverflow=on
  Sum4 : Sum  SaturateOnIntegerOverflow=on
  Sum5 : Sum  SaturateOnIntegerOverflow=on
  Switch1 : Switch  Threshold=0.5  SaturateOnIntegerOverflow=off  InputSameDT=off
  Switch2 : Switch  Threshold=0.5  SaturateOnIntegerOverflow=off  InputSameDT=off
  Unit Delay1 : UnitDelay  SampleTime=-1
  Unit Delay2 : UnitDelay  SampleTime=-1
  kp1 : Gain  Gain=CTRPIFF_CLIP_RELEASE*ts_inv  SaturateOnIntegerOverflow=on  OutDataTypeStr=Inherit: Same as input  ParamDataTypeStr=Inherit: Same as input
  kp2 : Gain  Gain=ki_i*ts_inv  SaturateOnIntegerOverflow=on  OutDataTypeStr=Inherit: Same as input  ParamDataTypeStr=Inherit: Same as input
  Vqs_out : Outport  VectorParamsAs1DForOutWhenUnconnected=off
  wires:
  Constant/1 -> Switch2/1
  [clip] -> Switch1/2
  [clip] -> Switch2/2
  clip/1 -> Unit Delay1/1
  kp2/1 -> Switch2/3
  Switch2/1 -> Sum4/1
  1/Ti/1 -> Sum5/1
  Unit Delay2/1 -> Sum2/1, kp1/1, Sum4/2
  Sum2/1 -> Switch1/1
  kp1/1 -> Sum2/2
  Sum4/1 -> Sum5/2, Switch1/3
  Switch1/1 -> Unit Delay2/1
  iq_tilde/1 -> 1/Ti/1, kp2/1
  Unit Delay1/1 -> [clip]
  Sum5/1 -> Vqs_out/1

== system psm_sv_ekf_bemf_ctrl/inv_psm_mod1/inverter_ctrl/inverter_control/current_ctrl/current_ctrl/dq_pi_with_vector_antiwindup mod1/dq_vector_pi/switch ==
  clip 1 : Inport
  clip 2 : Inport  Port=2
  Constant4 : Constant
  Constant5 : Constant  Value=0
  Sum1 : Sum  SaturateOnIntegerOverflow=on
  Switch : Switch  Threshold=0.5  SaturateOnIntegerOverflow=off  InputSameDT=off
  clip : Outport  VectorParamsAs1DForOutWhenUnconnected=off
  wires:
  Constant5/1 -> Switch/3
  Switch/1 -> clip/1
  Constant4/1 -> Switch/1
  Sum1/1 -> Switch/2
  clip 1/1 -> Sum1/1
  clip 2/1 -> Sum1/2

== system psm_sv_ekf_bemf_ctrl/inv_psm_mod1/inverter_ctrl/inverter_control/current_ctrl/current_ctrl/dq_pi_with_vector_antiwindup mod1/dq_vector_pi/vector lenght ==
  md : Inport
  mq : Inport  Port=2
  Math Function : Math  Operator=magnitude^2  SignedPower=on
  Math Function1 : Math  Operator=magnitude^2  SignedPower=on
  Math Function2 : Math  Operator=reciprocal  SignedPower=on
  Sqrt : Sqrt
  Sum5 : Sum  SaturateOnIntegerOverflow=on
  m_1 : Outport  VectorParamsAs1DForOutWhenUnconnected=off
  m : Outport  Port=2  VectorParamsAs1DForOutWhenUnconnected=off
  wires:
  Sqrt/1 -> m/1, Math Function2/1
  mq/1 -> Math Function1/1
  Math Function1/1 -> Sum5/2
  Math Function/1 -> Sum5/1
  Sum5/1 -> Sqrt/1
  Math Function2/1 -> m_1/1
  md/1 -> Math Function/1

== system psm_sv_ekf_bemf_ctrl/inv_psm_mod1/inverter_ctrl/inverter_control/current_ctrl/current_ctrl/dq_pi_with_vector_antiwindup mod1/dq_vector_pi_ccaller/Reset ==
  Step : Step  Time=0.05  InitialValue=1  FinalValue=0
  en : Outport
  wires:
  Step/1 -> en/1

== matlab function psm_sv_ekf_bemf_ctrl/inv_psm_mod1/inverter_ctrl/inverter_control/current_ctrl/current_ctrl/output voltage transformation/dq2alphabeta ==
  data: d input; alpha output; q input; gamma input; beta output
function [alpha,beta] = dq2alphabeta(d,q,gamma)

    alpha  =  d*cos(gamma) - q*sin(gamma);
    beta = d*sin(gamma) + q*cos(gamma);

end

== matlab function psm_sv_ekf_bemf_ctrl/inv_psm_mod1/inverter/timer/MATLAB Function ==
  data: t input; y output; phase input; period input
function y = ramp_up_down(t,phase,period)
x = sin(2*pi/period*t - phase -pi/2);
y = asin(x)/pi + 1/2;

== matlab function psm_sv_ekf_bemf_ctrl/inv_psm_mod1/inverter_ctrl/inverter_control/encoder-sensorless-switch/double_integrator_observer/bounder1 ==
  data: u input; y output
function y = bounder(u)
    y = -pi + mod(u+3*pi,2*pi);
end

== matlab function psm_sv_ekf_bemf_ctrl/inv_psm_mod1/inverter_ctrl/inverter_control/encoder-sensorless-switch/double_integrator_observer/bounder2 ==
  data: u input; y output
function y = bounder(u)
    y = -pi + mod(u+3*pi,2*pi);
end

== matlab function psm_sv_ekf_bemf_ctrl/inv_psm_mod1/inverter_ctrl/inverter_control/current_ctrl/EKF_bemf_observer/extended_kalman_observer/double_integrator_observer/bounder1 ==
  data: u input; y output
function y = bounder(u)
    y = -pi + mod(u+3*pi,2*pi);
end

== matlab function psm_sv_ekf_bemf_ctrl/inv_psm_mod1/inverter/MATLAB Function ==
  data: ua input; uu output; uv output; uw output; ub input
function [uu, uv, uw] = ab2uvw(ua, ub)

uu = ua;
uv = -ua/2 + sqrt(3)/2*ub;
uw = -ua/2 - sqrt(3)/2*ub;

== matlab function psm_sv_ekf_bemf_ctrl/inv_psm_mod1/inverter_ctrl/inverter_control/encoder-sensorless-switch/MATLAB Function ==
  data: omega_ctrl output; phase_psm input; omega_obs input; phase_obs input; phase_ctrl output; omega_psm input; omega_th parameter
function [omega_ctrl, phase_ctrl] = switch_enc2obs(phase_psm, omega_obs, phase_obs, omega_psm, omega_th)

if abs(omega_psm) > omega_th
    omega_ctrl = omega_obs;
    phase_ctrl = phase_obs;
else
    omega_ctrl = omega_psm;
    phase_ctrl = phase_psm;
end

== matlab function psm_sv_ekf_bemf_ctrl/inv_psm_mod1/inverter_ctrl/inverter_control/current_ctrl/EKF_bemf_observer/extended_kalman_observer/double_integrator_observer/bounder2 ==
  data: u input; y output
function y = bounder(u)
    y = -pi + mod(u+3*pi,2*pi);
end

== matlab function psm_sv_ekf_bemf_ctrl/inv_psm_mod1/inverter_ctrl/inverter_control/current_ctrl/current_transformation/alphabeta2dq ==
  data: alpha input; d output; beta input; gamma input; q output
function [d,q] = alphabeta2dq(alpha,beta,gamma)

    d  =  alpha*cos(gamma) + beta*sin(gamma);
    q = -alpha*sin(gamma) + beta*cos(gamma);

end

== matlab function psm_sv_ekf_bemf_ctrl/inv_psm_mod1/inverter_ctrl/inverter_control/current_ctrl/current_transformation/uvw2alphabeta ==
  data: u input; alpha output; v input; w input; beta output
function [alpha,beta] = uvw2alphabeta(u,v,w)

alpha = 2/3*(u - 1/2*v - 1/2*w);
beta  = 2/3*(sqrt(3)/2*(v - w));

end
